simulink library "rigidBody_lib"  (R2018b)
settings: Solver=VariableStepAuto  StartTime=0.0  StopTime=10.0  RelTol=1e-3
undefined symbols (not defined in the file or in its folder): quad
libraries: axes_transformation_lib x4, $bdroot x3
settings Model: Creator=Ybeyer  LastModifiedBy=yannic
settings DebuggingCC: LibraryContextMissingDiagnostic=none
settings SFSimCC: SimUseLocalCustomCode=off
settings RTWCC: RTWUseLocalCustomCode=off
settings CodeAppCC: StateflowObjectComments=on

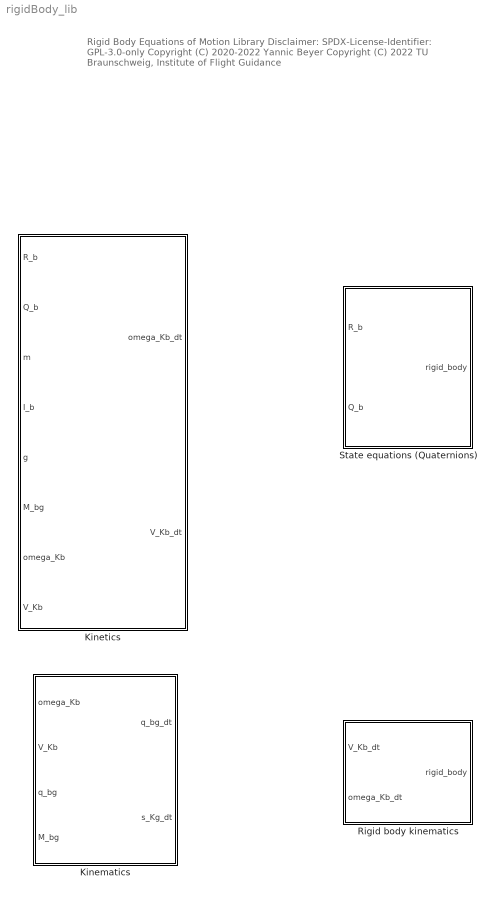
== system rigidBody_lib ==
  note: Rigid Body Equations of Motion Library
      |
      | Disclaimer:
      | SPDX-License-Identifier: GPL-3.0-only
      |
      | Copyright (C) 2020-2022 Yannic Beyer
      | Copyright (C) 2022 TU Braunschweig, Institute of Flight Guidance
  Kinematics : Subsystem
      mask Help: web('https://github.com/iff-gsc/LADAC/blob/main/equations_of_motion/rigid_body/README.md','-browser')
      mask DialogControl DescGroupVar Prompt: Kinematics
      mask DialogControl DescTextVar Prompt: This block calls the kinematics function and reshapes the signals to assure column vectors.
      mask DialogControl Control2 Prompt: More info can be found in the README:
      mask DialogControl Control3 Prompt: README
      mask DialogControl Control3 Callback: web('https://github.com/iff-gsc/LADAC/blob/main/equations_of_motion/rigid_body/README.md','-browser')
  Kinetics : Subsystem
      mask Help: web('https://github.com/iff-gsc/LADAC/blob/main/equations_of_motion/rigid_body/README.md','-browser')
      mask DialogControl DescGroupVar Prompt: Kinetics
      mask DialogControl DescTextVar Prompt: This block calls the kinetics function and reshapes the signals to assure column vectors.
      mask DialogControl Control2 Prompt: More info can be found in the README:
      mask DialogControl Control3 Prompt: README
      mask DialogControl Control3 Callback: web('https://github.com/iff-gsc/LADAC/blob/main/equations_of_motion/rigid_body/README.md','-browser')
  Rigid body kinematics : Subsystem  mask{omega_Kb_0=[0;0;0], q_bg_0=[1;0;0;0], V_Kb_0=[0;0;0], s_g_0=[0;0;0]}
      mask prompts: omega_Kb_0 "initial angular velocity vector, 1/s"; q_bg_0 "initial quaternions vector"; V_Kb_0 "initial velocity vector, m/s"; s_g_0 "initial position vector, m"
      mask Help: web('https://github.com/iff-gsc/LADAC/blob/main/equations_of_motion/rigid_body/README.md','-browser')
      mask DialogControl DescGroupVar Prompt: Rigid Body kinematics
      mask DialogControl DescTextVar Prompt: More info can be found in the README:
      mask DialogControl Control3 Prompt: README
      mask DialogControl Control3 Callback: web('https://github.com/iff-gsc/LADAC/blob/main/equations_of_motion/rigid_body/README.md','-browser')
  State equations (Quaternions) : Subsystem  mask{m=1, I=eye(3), is_g_checked=off, g=10, omega_Kb_0=[0,0,0]', q_bg_0=[1,0,0,0]', V_Kb_0=[0,0,0]', s_g_0=[0,0,0]'}
      mask prompts: m "mass, kg"; I "inertia matrix, kg*m^2"; is_g_checked "enable external gravitational acceleration"; g "earth acceleration, m/s^2"; omega_Kb_0 "initial rate vector, 1/s"; q_bg_0 "initial quaternions vector"; V_Kb_0 "initial velocity vector"; s_g_0 "initial position vector"
      mask init:
      | rigidBodyBlockInit(is_g_checked);
      mask Help: web('https://github.com/iff-gsc/LADAC/blob/main/equations_of_motion/rigid_body/README.md','-browser')
      mask DialogControl DescGroupVar Prompt: State equations (Quaternions)
      mask DialogControl Control3 Prompt: More info can be found in the README:
      mask DialogControl Control4 Prompt: README
      mask DialogControl Control4 Callback: web('https://github.com/iff-gsc/LADAC/blob/main/equations_of_motion/rigid_body/README.md','-browser')

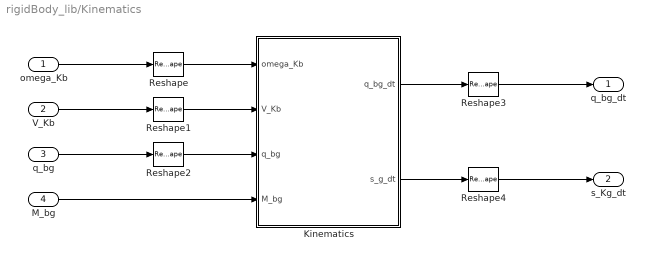
== system rigidBody_lib/Kinematics ==
  omega_Kb : Inport
  V_Kb : Inport  Port=2
  q_bg : Inport  Port=3
  M_bg : Inport  Port=4
  Kinematics : MATLAB Function  TreatAsAtomicUnit=on
  Reshape{,1..4} (5 alike) : Reshape  OutputDimensionality=Column vector (2-D)
  q_bg_dt : Outport
  s_Kg_dt : Outport  Port=2
  wires:
  omega_Kb/1 -> Reshape/1
  Kinematics/1(q_bg_dt) -> Reshape3/1
  Kinematics/2(s_g_dt) -> Reshape4/1
  M_bg/1 -> Kinematics/4(M_bg)
  V_Kb/1 -> Reshape1/1
  q_bg/1 -> Reshape2/1
  Reshape/1 -> Kinematics/1(omega_Kb)
  Reshape1/1 -> Kinematics/2(V_Kb)
  Reshape2/1 -> Kinematics/3(q_bg)
  Reshape3/1 -> q_bg_dt/1
  Reshape4/1 -> s_Kg_dt/1

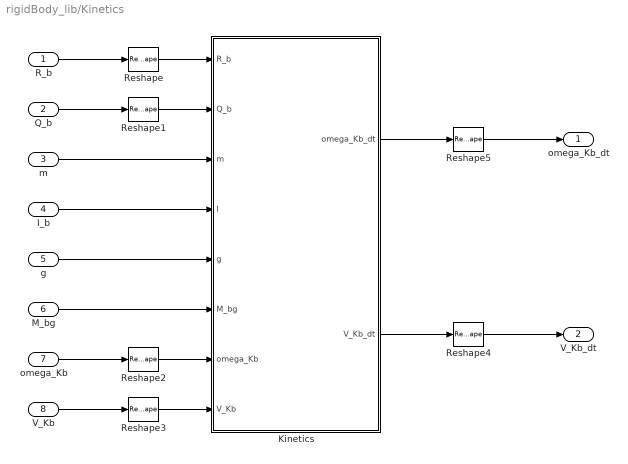
== system rigidBody_lib/Kinetics ==
  R_b : Inport
  Q_b : Inport  Port=2
  m : Inport  Port=3
  I_b : Inport  Port=4
  g : Inport  Port=5
  M_bg : Inport  Port=6
  omega_Kb : Inport  Port=7
  V_Kb : Inport  Port=8
  Kinetics : MATLAB Function  TreatAsAtomicUnit=on
  Reshape{,1..5} (6 alike) : Reshape  OutputDimensionality=Column vector (2-D)
  omega_Kb_dt : Outport
  V_Kb_dt : Outport  Port=2
  wires:
  m/1 -> Kinetics/3(m)
  V_Kb/1 -> Reshape3/1
  I_b/1 -> Kinetics/4(I)
  omega_Kb/1 -> Reshape2/1
  Q_b/1 -> Reshape1/1
  R_b/1 -> Reshape/1
  Kinetics/2(V_Kb_dt) -> Reshape4/1
  M_bg/1 -> Kinetics/6(M_bg)
  Kinetics/1(omega_Kb_dt) -> Reshape5/1
  g/1 -> Kinetics/5(g)
  Reshape/1 -> Kinetics/1(R_b)
  Reshape1/1 -> Kinetics/2(Q_b)
  Reshape2/1 -> Kinetics/7(omega_Kb)
  Reshape3/1 -> Kinetics/8(V_Kb)
  Reshape4/1 -> V_Kb_dt/1
  Reshape5/1 -> omega_Kb_dt/1

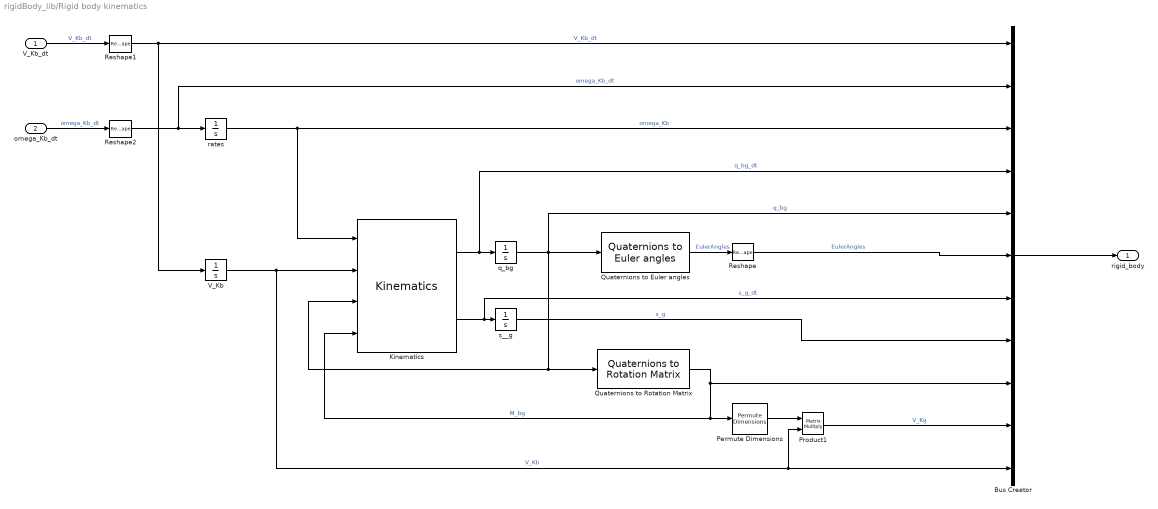
== system rigidBody_lib/Rigid body kinematics ==
  V_Kb_dt : Inport
  omega_Kb_dt : Inport  Port=2
  Bus Creator : BusCreator  Inputs=11
  Kinematics : $bdroot/Kinematics
  Permute Dimensions : PermuteDimensions
  Product1 : Product  Multiplication=Matrix(*)
  Quaternions to Euler angles : axes_transformation_lib/Quaternions to Euler angles  SystemSampleTime=-1
      settings: SourceProductName=LADAC
  Quaternions to Rotation Matrix : axes_transformation_lib/Quaternions to Rotation Matrix  SystemSampleTime=-1
      settings: SourceProductName=LADAC
  Reshape : Reshape  OutputDimensionality=Column vector (2-D)
  Reshape1 : Reshape  OutputDimensionality=Column vector (2-D)
  Reshape2 : Reshape  OutputDimensionality=Column vector (2-D)
  V_Kb : Integrator  InitialCondition=V_Kb_0  ContinuousStateAttributes='velocity'
  q_bg : Integrator  InitialCondition=q_bg_0  UpperSaturationLimit=[inf;inf;-quad.z_s]  LowerSaturationLimit=[-inf;-inf;-inf]  ContinuousStateAttributes='quaternion'
  rates : Integrator  InitialCondition=omega_Kb_0  ContinuousStateAttributes='rates'
  s__g : Integrator  InitialCondition=s_g_0  UpperSaturationLimit=[inf;inf;-quad.z_s]  LowerSaturationLimit=[-inf;-inf;-inf]  ContinuousStateAttributes='position'
  rigid_body : Outport
  wires:
  Bus Creator/1 -> rigid_body/1
  Kinematics/2 -> Bus Creator/7, s__g/1  "s_g_dt"
  Permute Dimensions/1 -> Product1/1
  Quaternions to Rotation Matrix/1 -> Kinematics/4, Permute Dimensions/1, Bus Creator/9  "M_bg"
  Quaternions to Euler angles/1 -> Reshape/1  "EulerAngles"
  q_bg/1 -> Kinematics/3, Quaternions to Rotation Matrix/1, Bus Creator/5, Quaternions to Euler angles/1  "q_bg"
  V_Kb/1 -> Kinematics/2, Product1/2, Bus Creator/11  "V_Kb"
  Kinematics/1 -> Bus Creator/4, q_bg/1  "q_bg_dt"
  s__g/1 -> Bus Creator/8  "s_g"
  rates/1 -> Kinematics/1, Bus Creator/3  "omega_Kb"
  omega_Kb_dt/1 -> Reshape2/1  "omega_Kb_dt"
  V_Kb_dt/1 -> Reshape1/1  "V_Kb_dt"
  Product1/1 -> Bus Creator/10  "V_Kg"
  Reshape/1 -> Bus Creator/6  "EulerAngles"
  Reshape1/1 -> V_Kb/1, Bus Creator/1  "V_Kb_dt"
  Reshape2/1 -> Bus Creator/2, rates/1  "omega_Kb_dt"

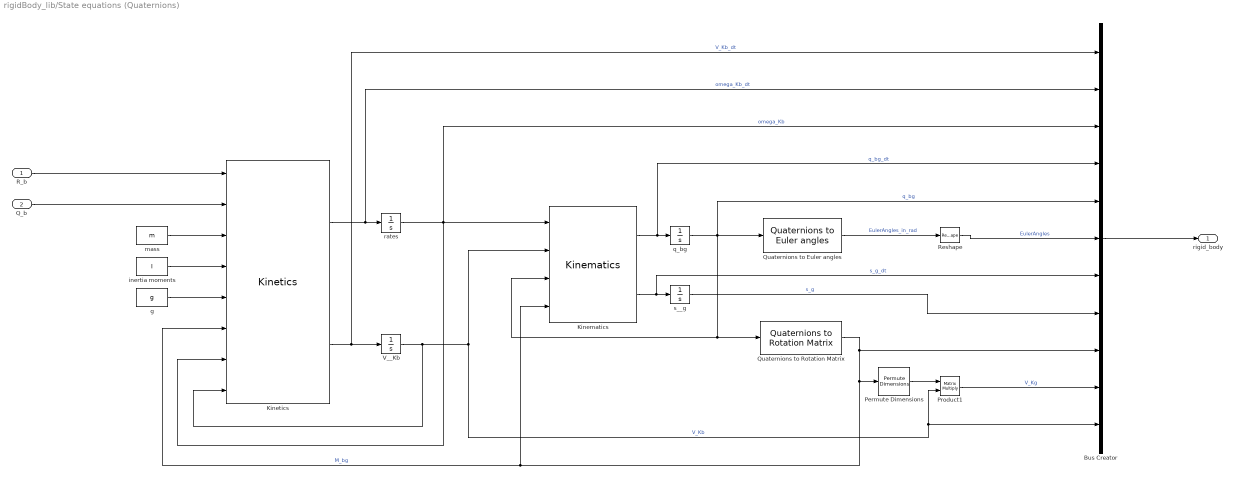
== system rigidBody_lib/State equations (Quaternions) ==
  R_b : Inport  PortDimensions=3
  Q_b : Inport  Port=2  PortDimensions=3
  Bus Creator : BusCreator  Inputs=11
  Kinematics : $bdroot/Kinematics
  Kinetics : $bdroot/Kinetics
  Permute Dimensions : PermuteDimensions
  Product1 : Product  Multiplication=Matrix(*)
  Quaternions to Euler angles : axes_transformation_lib/Quaternions to Euler angles  SystemSampleTime=-1
      settings: SourceProductName=LADAC
  Quaternions to Rotation Matrix : axes_transformation_lib/Quaternions to Rotation Matrix  SystemSampleTime=-1
      settings: SourceProductName=LADAC
  Reshape : Reshape  OutputDimensionality=Column vector (2-D)
  V__Kb : Integrator  InitialCondition=V_Kb_0  ContinuousStateAttributes='velocity'
  g : Constant  Value=g
  inertia moments : Constant  Value=I
  mass : Constant  Value=m
  q_bg : Integrator  InitialCondition=q_bg_0  UpperSaturationLimit=[inf;inf;-quad.z_s]  LowerSaturationLimit=[-inf;-inf;-inf]  ContinuousStateAttributes='quaternion'
  rates : Integrator  InitialCondition=omega_Kb_0  ContinuousStateAttributes='rates'
  s__g : Integrator  InitialCondition=s_g_0  UpperSaturationLimit=[inf;inf;-quad.z_s]  LowerSaturationLimit=[-inf;-inf;-inf]  ContinuousStateAttributes='position'
  rigid_body : Outport
  wires:
  inertia moments/1 -> Kinetics/4
  Kinetics/1 -> Bus Creator/2, rates/1  "omega_Kb_dt"
  g/1 -> Kinetics/5
  R_b/1 -> Kinetics/1
  mass/1 -> Kinetics/3
  Kinetics/2 -> Bus Creator/1, V__Kb/1  "V_Kb_dt"
  s__g/1 -> Bus Creator/8  "s_g"
  V__Kb/1 -> Kinetics/8, Kinematics/2, Product1/2, Bus Creator/11  "V_Kb"
  Kinematics/2 -> Bus Creator/7, s__g/1  "s_g_dt"
  Kinematics/1 -> Bus Creator/4, q_bg/1  "q_bg_dt"
  q_bg/1 -> Bus Creator/5, Quaternions to Euler angles/1, Kinematics/3, Quaternions to Rotation Matrix/1  "q_bg"
  Quaternions to Euler angles/1 -> Reshape/1  "EulerAngles_in_rad"
  Q_b/1 -> Kinetics/2
  Quaternions to Rotation Matrix/1 -> Permute Dimensions/1, Kinematics/4, Kinetics/6, Bus Creator/9  "M_bg"
  rates/1 -> Kinematics/1, Kinetics/7, Bus Creator/3  "omega_Kb"
  Product1/1 -> Bus Creator/10  "V_Kg"
  Permute Dimensions/1 -> Product1/1
  Bus Creator/1 -> rigid_body/1
  Reshape/1 -> Bus Creator/6  "EulerAngles"

== matlab function rigidBody_lib/Kinetics/Kinetics ==
  data: R_b input; Q_b input; m input; I input; g input; M_bg input; omega_Kb input; V_Kb input; omega_Kb_dt output; V_Kb_dt output
function [omega_Kb_dt, V_Kb_dt] = ...
    fcn( R_b, Q_b, m, I, g, M_bg, omega_Kb, V_Kb )%#codegen
[omega_Kb_dt, V_Kb_dt] = ...
    rigidBodyKinetics( R_b, Q_b, m, I, g, M_bg, omega_Kb, V_Kb );

== matlab function rigidBody_lib/Kinematics/Kinematics ==
  data: omega_Kb input; q_bg_dt output; V_Kb input; q_bg input; s_g_dt output; M_bg input
function [q_bg_dt, s_g_dt] = ...
    fcn( omega_Kb, V_Kb, q_bg, M_bg )%#codegen
[q_bg_dt, s_g_dt] = ...
    rigidBodyKinematicsQuat( omega_Kb, V_Kb, q_bg, M_bg );
